simulink model "My_gfm_battery_sil_1_BS_4_2"  (R2018b)
settings: Solver=ode23t  StartTime=0.0  StopTime=30  MaxStep=1e-4  RelTol=1e-3
PreLoadFcn:
  | modelDir = fileparts(get_param(bdroot,'FileName'));
  | 
  | load_system(fullfile(modelDir,'controls_element_lib.slx'));
  | load_system(fullfile(modelDir,'test_sequence_lib.slx'));
InitFcn:
  | close all;
  | clear all;
  | clc;
  | 
  | % frequency nominals
  | F_NOM = 60;
  | W_NOM = 2 * pi * F_NOM;
  | 
  | % base values relative to inverter
  | % --------------------------------
  | VLL_INV_NOM = 480;
  | P_INV_NOM = 1e6;
  | Q_INV_NOM = 0.5e6;
  | S_INV_NOM = sqrt(P_INV_NOM^2 + Q_INV_NOM^2);
  | 
  | I_INV_BASE = S_INV_NOM/(sqrt(3)*VLL_INV_NOM);
  | Z_INV_BASE = VLL_INV_NOM^2/S_INV_NOM;
  | L_INV_BASE = Z_INV_BASE / W_NOM;
  | C_INV_BASE = 1 / (Z_INV_BASE * W_NOM);
  | 
  | % nominal ratings for power system model
  | % --------------------------------------
  | INVERTER_COUNT = 100;
  | 
  | VLV_NOM = VLL_INV_NOM;
  | VMV_NOM = 35e3;
  | VHV_NOM = 230e3;
  | S_PLANT = INVERTER_COUNT * S_INV_NOM;
  | 
  | N_GSU = VHV_NOM/VMV_NOM;
  | N_MVT = VMV_NOM/VLV_NOM;
  | 
  | I_LV_BASE = S_PLANT/(sqrt(3)*VLV_NOM);
  | I_MV_BASE = S_PLANT/(sqrt(3)*VMV_NOM);
  | I_HV_BASE = S_PLANT/(sqrt(3)*VHV_NOM);
  | 
  | Z_LV_BASE = VLV_NOM^2/S_PLANT;
  | Z_MV_BASE = VMV_NOM^2/S_PLANT;
  | Z_HV_BASE = VHV_NOM^2/S_PLANT;
  | 
  | L_LV_BASE = Z_LV_BASE / W_NOM;
  | L_MV_BASE = Z_MV_BASE / W_NOM;
  | L_HV_BASE = Z_HV_BASE / W_NOM;
  | C_LV_BASE = 1 / (Z_LV_BASE * W_NOM);
  | C_MV_BASE = 1 / (Z_MV_BASE * W_NOM);
  | C_HV_BASE = 1 / (Z_HV_BASE * W_NOM);
undefined symbols (not defined in the file): j
libraries: simulink x54, test_sequence_lib x9, controls_element_lib x7
(part 6 of 6)

== system My_gfm_battery_sil_1_BS_4_2/My Inverter Controller /My_machineModel_Other Exciter/power analyzer ==
  iac : Inport
  vac : Inport  Port=2
  Demux1 : Demux  Outputs=3
  Demux2 : Demux  Outputs=3
  Gain3 : Gain  Gain=1 / sqrt(3)
  Product{,1..3} (4 alike) : Product
  Sum of Elements : Sum  Inputs=+
  Sum2 : Sum  Inputs=|+-
  Sum3 : Sum  Inputs=|+-
  Sum4 : Sum  Inputs=|+-
  Sum5 : Sum  Inputs=+++
  P : Outport  VectorParamsAs1DForOutWhenUnconnected=on
  Q : Outport  Port=2  VectorParamsAs1DForOutWhenUnconnected=on
  wires:
  Product/1 -> Sum of Elements/1
  Sum of Elements/1 -> P/1  "P"
  Gain3/1 -> Q/1  "Q"
  Demux1/1 -> Product2/2  "ia"
  Demux2/1 -> Sum2/1, Sum4/2
  Sum2/1 -> Product1/1  "vab"
  Sum5/1 -> Gain3/1
  Sum3/1 -> Product2/1  "vbc"
  iac/1 -> Demux1/1, Product/1
  vac/1 -> Product/2, Demux2/1
  Demux1/2 -> Product3/2  "ib"
  Demux1/3 -> Product1/2  "ic"
  Demux2/3 -> Sum3/2, Sum4/1
  Demux2/2 -> Sum2/2, Sum3/1
  Product3/1 -> Sum5/2
  Sum4/1 -> Product3/1  "vca"
  Product2/1 -> Sum5/3
  Product1/1 -> Sum5/1

== system My_gfm_battery_sil_1_BS_4_2/My Inverter Controller /My_machineModel_Other Exciter/rotor model ==
  p_mechanical : Inport
  p_electrical : Inport  Port=2
  Constant : Constant  Value=nominalFrequency
  HPF (wDamperDecoupler) : TransferFcn  Commented=on  Numerator=[0.3 0]  Denominator=[0.3 1]
  HPF (wDamperDecoupler) 1 : Subsystem
  Integrator1 : Integrator  LimitOutput=on  UpperSaturationLimit=5  LowerSaturationLimit=-5
  Sum : Sum  Inputs=++|
  Sum2 : Sum  Inputs=|+-
  Sum3 : Sum  Inputs=|+-
  k_damp : Gain  Gain=kDamper*SRated
  k_inertia : Gain  Gain=(nominalFrequency/2)/(inertialConstant*SRated)
  oscillator_3ph : Subsystem
  osc[3] : Outport  VectorParamsAs1DForOutWhenUnconnected=on
  f_rotor : Outport  Port=2  VectorParamsAs1DForOutWhenUnconnected=on
  wires:
  Constant/1 -> Sum/1
  Sum/1 -> oscillator_3ph/1(f), f_rotor/1
  k_damp/1 -> Sum2/2
  Integrator1/1 -> HPF (wDamperDecoupler) 1/1(in), Sum/2
  p_mechanical/1 -> Sum3/1
  Sum3/1 -> Sum2/1
  p_electrical/1 -> Sum3/2
  HPF (wDamperDecoupler) 1/1(out) -> k_damp/1
  oscillator_3ph/1(osc[3]) -> osc[3]/1
  k_inertia/1 -> Integrator1/1
  Sum2/1 -> k_inertia/1

== system My_gfm_battery_sil_1_BS_4_2/My Inverter Controller /My_machineModel_Other Exciter/voltage analyzer ==
  osc[3] : Inport
  v_terminal : Inport  Port=2
  Complex to Magnitude-Angle : ComplexToMagnitudeAngle
  Complex to Real-Imag : ComplexToRealImag
  Conj : Math  Operator=conj  SaturateOnIntegerOverflow=on
  LPF : Subsystem
  "LPF " : Subsystem
  Product1 : Product
  Product2 : Product
  Real-Imag to Complex1 : RealImagToComplex
  Sum of Elements1 : Sum  Inputs=+
  Sum of Elements2 : Sum  Inputs=+
  Terminator : Terminator
  over_sqrt(3) : Gain  Gain=1/sqrt(3)
  over_sqrt(3)1 : Gain  Gain=1/sqrt(3)
  sqrt(2) : Gain  Gain=sqrt(2)
  Vd : Outport  VectorParamsAs1DForOutWhenUnconnected=on
  Vq : Outport  Port=2  VectorParamsAs1DForOutWhenUnconnected=on
  Vt_Mag : Outport  Port=3  VectorParamsAs1DForOutWhenUnconnected=on
  wires:
  "LPF "/1(Out) -> Real-Imag to Complex1/2, Vq/1  "Vq"
  osc[3]/1 -> Conj/1
  LPF/1(Out) -> Real-Imag to Complex1/1, Vd/1  "Vd"
  over_sqrt(3)1/1 -> LPF/1(In)
  over_sqrt(3)/1 -> "LPF "/1(In)
  Complex to Real-Imag/1 -> Product2/1
  Complex to Real-Imag/2 -> Product1/1
  Sum of Elements2/1 -> over_sqrt(3)1/1
  v_terminal/1 -> Product2/2, Product1/2
  Product1/1 -> Sum of Elements1/1
  Sum of Elements1/1 -> over_sqrt(3)/1
  sqrt(2)/1 -> Complex to Real-Imag/1
  Conj/1 -> sqrt(2)/1
  Product2/1 -> Sum of Elements2/1
  Complex to Magnitude-Angle/1 -> Vt_Mag/1  "Vt"
  Real-Imag to Complex1/1 -> Complex to Magnitude-Angle/1  "Vd"
  Complex to Magnitude-Angle/2 -> Terminator/1

== system My_gfm_battery_sil_1_BS_4_2/My Inverter Controller /modesAndProtection_A/hardware_protection ==
  vdc : Inport
  Clear Timer : Subsystem  mask{T_STEP=1e-3, TIMEOUT=dcTripClearTimeout}
      mask prompts: T_STEP "Time step"
  Compare To Constant1 : simulink/Logic and Bit Operations/Compare To Constant  relop=<  const=dcUndervotlageThreshold  OutDataTypeStr=boolean
  Compare To Constant2 : simulink/Logic and Bit Operations/Compare To Constant  relop=>  const=dcOvervotlageThreshold  OutDataTypeStr=boolean
  NOT : Logic  Operator=NOT  IconShape=distinctive  AllPortsSameDT=off  OutDataTypeStr=boolean
  OR : Logic  Operator=OR  IconShape=distinctive  AllPortsSameDT=off  OutDataTypeStr=boolean
  Zero-Order Hold1 : ZeroOrderHold  SampleTime=200e-6
  all_clear : Outport  VectorParamsAs1DForOutWhenUnconnected=on
  wires:
  NOT/1 -> all_clear/1
  Zero-Order Hold1/1 -> Compare To Constant2/1, Compare To Constant1/1
  Compare To Constant2/1 -> OR/1  "dcOV"
  Clear Timer/1(out) -> NOT/1
  OR/1 -> Clear Timer/1(in)
  Compare To Constant1/1 -> OR/2  "dcUV"
  vdc/1 -> Zero-Order Hold1/1

== system My_gfm_battery_sil_1_BS_4_2/Plant controller (simplified example)1/LVRT_foldback/LPF ==
  in : Inport
  1/0.01 : Gain  Gain=1/0.01
  Integrator : Integrator
  Sum3 : Sum  Inputs=|+-
  out : Outport  VectorParamsAs1DForOutWhenUnconnected=on
  wires:
  Integrator/1 -> out/1, Sum3/2
  Sum3/1 -> 1/0.01/1
  in/1 -> Sum3/1
  1/0.01/1 -> Integrator/1

== system My_gfm_battery_sil_1_BS_4_2/Plant controller (simplified example)1/LVRT_foldback/assymmetric filter ==
  in : Inport
  Gain1 : Gain  Gain=1/0.01
  Integrator : Integrator
  Saturation1 : Saturate  UpperLimit=0.05 * 1  LowerLimit=-1 * 1
  Sum3 : Sum  Inputs=|+-
  out : Outport  VectorParamsAs1DForOutWhenUnconnected=on
  wires:
  Integrator/1 -> out/1, Sum3/2
  Sum3/1 -> Saturation1/1
  in/1 -> Sum3/1
  Gain1/1 -> Integrator/1
  Saturation1/1 -> Gain1/1

== system My_gfm_battery_sil_1_BS_4_2/Plant controller (simplified example)1/Meter/PLL-analog ==
  note: cos x - j sin x
      | cos (x-120) - j (sin x -120)
      | cos (x+120) - j (sin x +120)
  note: cos x + j sin x
      | cos (x-120) + j (sin x -120)
      | cos (x+120) + j (sin x +120)
  note: -sin x
      |  -sin (x -120)
      |  -sin (x +120)
  note: cos x + j sin x
      | cos (x-120) + j (sin x -120)
      | cos (x+120) + j (sin x +120)
  ref : Inport
  Complex to Real-Imag : ComplexToRealImag
  Conj : Math  Operator=conj  SaturateOnIntegerOverflow=on
  Gain : Gain  Gain=3
  Gain2 : Gain  Gain=30
  Integrator : Integrator  LimitOutput=on  UpperSaturationLimit=5  LowerSaturationLimit=-5
  Product2 : Product
  Saturation : Saturate  UpperLimit=5  LowerLimit=-5
  Sum of Elements : Sum  Inputs=+
  Sum1 : Sum  Inputs=|++
  Sum2 : Sum  Inputs=|++
  Terminator : Terminator
  Transfer Fcn : TransferFcn  Denominator=[0.02 1]
  fnom : Constant  Value=60
  oscillator_3ph : Subsystem
  freq : Outport  VectorParamsAs1DForOutWhenUnconnected=on
  osc : Outport  Port=2  VectorParamsAs1DForOutWhenUnconnected=on
  wires:
  Gain2/1 -> Integrator/1
  Integrator/1 -> Sum2/2
  Sum2/1 -> Sum1/1
  fnom/1 -> Sum1/2
  Product2/1 -> Sum of Elements/1
  Transfer Fcn/1 -> Gain/1, Gain2/1
  Saturation/1 -> Sum2/1
  Gain/1 -> Saturation/1
  Sum1/1 -> oscillator_3ph/1(f), freq/1
  ref/1 -> Product2/1
  Sum of Elements/1 -> Transfer Fcn/1
  Conj/1 -> Complex to Real-Imag/1
  Complex to Real-Imag/1 -> Terminator/1
  Complex to Real-Imag/2 -> Product2/2
  oscillator_3ph/1(osc[3]) -> osc/1, Conj/1

== system My_gfm_battery_sil_1_BS_4_2/Plant controller (simplified example)1/VoltVAr/LPF ==
  in : Inport
  1/0.05 : Gain  Gain=1/0.05
  Integrator : Integrator
  Sum3 : Sum  Inputs=|+-
  out : Outport  VectorParamsAs1DForOutWhenUnconnected=on
  wires:
  Integrator/1 -> out/1, Sum3/2
  Sum3/1 -> 1/0.05/1
  in/1 -> Sum3/1
  1/0.05/1 -> Integrator/1

== system My_gfm_battery_sil_1_BS_4_2/Plant controller (simplified example)1/VoltVAr/LPF1 ==
  in : Inport
  1/0.05 : Gain  Gain=1/0.05
  1/0.1 : Gain
  Integrator : Integrator
  Saturation : Saturate  UpperLimit=inf  LowerLimit=0
  Saturation1 : Saturate  UpperLimit=0  LowerLimit=-inf
  Sum : Sum  Inputs=|++
  Sum3 : Sum  Inputs=|+-
  out : Outport  VectorParamsAs1DForOutWhenUnconnected=on
  wires:
  Integrator/1 -> out/1, Sum3/2
  Sum3/1 -> 1/0.1/1, 1/0.05/1
  in/1 -> Sum3/1
  1/0.05/1 -> Saturation/1
  Sum/1 -> Integrator/1
  1/0.1/1 -> Saturation1/1
  Saturation/1 -> Sum/1
  Saturation1/1 -> Sum/2

== system My_gfm_battery_sil_1_BS_4_2/Plant controller (simplified example)2/LVRT_foldback/LPF ==
  in : Inport
  1/0.01 : Gain  Gain=1/0.01
  Integrator : Integrator
  Sum3 : Sum  Inputs=|+-
  out : Outport  VectorParamsAs1DForOutWhenUnconnected=on
  wires:
  Integrator/1 -> out/1, Sum3/2
  Sum3/1 -> 1/0.01/1
  in/1 -> Sum3/1
  1/0.01/1 -> Integrator/1

== system My_gfm_battery_sil_1_BS_4_2/Plant controller (simplified example)2/LVRT_foldback/assymmetric filter ==
  in : Inport
  Gain1 : Gain  Gain=1/0.01
  Integrator : Integrator
  Saturation1 : Saturate  UpperLimit=0.05 * 1  LowerLimit=-1 * 1
  Sum3 : Sum  Inputs=|+-
  out : Outport  VectorParamsAs1DForOutWhenUnconnected=on
  wires:
  Integrator/1 -> out/1, Sum3/2
  Sum3/1 -> Saturation1/1
  in/1 -> Sum3/1
  Gain1/1 -> Integrator/1
  Saturation1/1 -> Gain1/1

== system My_gfm_battery_sil_1_BS_4_2/Plant controller (simplified example)2/Meter/PLL-analog ==
  note: cos x - j sin x
      | cos (x-120) - j (sin x -120)
      | cos (x+120) - j (sin x +120)
  note: cos x + j sin x
      | cos (x-120) + j (sin x -120)
      | cos (x+120) + j (sin x +120)
  note: -sin x
      |  -sin (x -120)
      |  -sin (x +120)
  note: cos x + j sin x
      | cos (x-120) + j (sin x -120)
      | cos (x+120) + j (sin x +120)
  ref : Inport
  en : Inport  Port=2
  Complex to Real-Imag : ComplexToRealImag
  Conj : Math  Operator=conj  SaturateOnIntegerOverflow=on
  Gain : Gain  Gain=3
  Gain2 : Gain  Gain=30
  Integrator : Integrator  ExternalReset=level  LimitOutput=on  UpperSaturationLimit=5  LowerSaturationLimit=-5
  Logical Operator : Logic  Operator=NOT  IconShape=distinctive  AllPortsSameDT=off  OutDataTypeStr=boolean
  Product2 : Product
  Saturation : Saturate  UpperLimit=5  LowerLimit=-5
  Sum of Elements : Sum  Inputs=+
  Sum1 : Sum  Inputs=|++
  Sum2 : Sum  Inputs=|++
  Terminator : Terminator
  Transfer Fcn : TransferFcn  Denominator=[0.02 1]
  fnom : Constant  Value=60
  oscillator_3ph : Subsystem
  freq : Outport  VectorParamsAs1DForOutWhenUnconnected=on
  osc : Outport  Port=2  VectorParamsAs1DForOutWhenUnconnected=on
  wires:
  Gain2/1 -> Integrator/1
  Integrator/1 -> Sum2/2
  Sum2/1 -> Sum1/1
  fnom/1 -> Sum1/2
  Product2/1 -> Sum of Elements/1
  Transfer Fcn/1 -> Gain/1, Gain2/1
  Saturation/1 -> Sum2/1
  Gain/1 -> Saturation/1
  Sum1/1 -> oscillator_3ph/1(f), freq/1
  ref/1 -> Product2/1
  Sum of Elements/1 -> Transfer Fcn/1
  Conj/1 -> Complex to Real-Imag/1
  Complex to Real-Imag/1 -> Terminator/1
  Complex to Real-Imag/2 -> Product2/2
  oscillator_3ph/1(osc[3]) -> osc/1, Conj/1
  en/1 -> Logical Operator/1
  Logical Operator/1 -> Integrator/2

== system My_gfm_battery_sil_1_BS_4_2/Plant controller (simplified example)2/Sync/LPF ==
  In : Inport
  1/0.02 : Gain  Gain=1/0.02
  Integrator : Integrator
  Sum3 : Sum  Inputs=|+-
  Out : Outport  VectorParamsAs1DForOutWhenUnconnected=on
  wires:
  Integrator/1 -> Out/1, Sum3/2
  Sum3/1 -> 1/0.02/1
  In/1 -> Sum3/1
  1/0.02/1 -> Integrator/1

== system My_gfm_battery_sil_1_BS_4_2/Plant controller (simplified example)2/Sync/LPF1 ==
  In : Inport
  1/0.02 : Gain  Gain=1/0.02
  Integrator : Integrator
  Sum3 : Sum  Inputs=|+-
  Out : Outport  VectorParamsAs1DForOutWhenUnconnected=on
  wires:
  Integrator/1 -> Out/1, Sum3/2
  Sum3/1 -> 1/0.02/1
  In/1 -> Sum3/1
  1/0.02/1 -> Integrator/1

== system My_gfm_battery_sil_1_BS_4_2/Plant controller (simplified example)2/VoltVAr/LPF ==
  in : Inport
  1/0.05 : Gain  Gain=1/0.05
  Integrator : Integrator
  Sum3 : Sum  Inputs=|+-
  out : Outport  VectorParamsAs1DForOutWhenUnconnected=on
  wires:
  Integrator/1 -> out/1, Sum3/2
  Sum3/1 -> 1/0.05/1
  in/1 -> Sum3/1
  1/0.05/1 -> Integrator/1

== system My_gfm_battery_sil_1_BS_4_2/Plant controller (simplified example)2/VoltVAr/LPF1 ==
  in : Inport
  1/0.05 : Gain  Gain=1/0.05
  1/0.1 : Gain
  Integrator : Integrator
  Saturation : Saturate  UpperLimit=inf  LowerLimit=0
  Saturation1 : Saturate  UpperLimit=0  LowerLimit=-inf
  Sum : Sum  Inputs=|++
  Sum3 : Sum  Inputs=|+-
  out : Outport  VectorParamsAs1DForOutWhenUnconnected=on
  wires:
  Integrator/1 -> out/1, Sum3/2
  Sum3/1 -> 1/0.1/1, 1/0.05/1
  in/1 -> Sum3/1
  1/0.05/1 -> Saturation/1
  Sum/1 -> Integrator/1
  1/0.1/1 -> Saturation1/1
  Saturation/1 -> Sum/1
  Saturation1/1 -> Sum/2

== system My_gfm_battery_sil_1_BS_4_2/My Inverter Controller /My_acMonitor_A/Analyzer_V/complex_LPF ==
  note: This was needed because Simulink complains when using transfer functions directly on arrays or complex numbers.
  In1 : Inport
  Complex to Real-Imag : ComplexToRealImag
  Gain2 : Gain  Gain=1/tau
  Gain3 : Gain  Gain=1/tau
  Integrator : Integrator
  Integrator1 : Integrator
  Real-Imag to Complex : RealImagToComplex
  Sum : Sum  Inputs=|+-
  Sum1 : Sum  Inputs=|+-
  Out1 : Outport  VectorParamsAs1DForOutWhenUnconnected=on
  wires:
  Real-Imag to Complex/1 -> Out1/1
  In1/1 -> Complex to Real-Imag/1
  Complex to Real-Imag/1 -> Sum/1
  Integrator/1 -> Real-Imag to Complex/1, Sum/2
  Sum1/1 -> Gain3/1
  Complex to Real-Imag/2 -> Sum1/1
  Gain2/1 -> Integrator/1
  Sum/1 -> Gain2/1
  Integrator1/1 -> Sum1/2, Real-Imag to Complex/2
  Gain3/1 -> Integrator1/1

== system My_gfm_battery_sil_1_BS_4_2/My Inverter Controller /My_acMonitor_A/Analyzer_V1/complex_LPF ==
  note: This was needed because Simulink complains when using transfer functions directly on arrays or complex numbers.
  In1 : Inport
  Complex to Real-Imag : ComplexToRealImag
  Gain2 : Gain  Gain=1/tau
  Gain3 : Gain  Gain=1/tau
  Integrator : Integrator
  Integrator1 : Integrator
  Real-Imag to Complex : RealImagToComplex
  Sum : Sum  Inputs=|+-
  Sum1 : Sum  Inputs=|+-
  Out1 : Outport  VectorParamsAs1DForOutWhenUnconnected=on
  wires:
  Real-Imag to Complex/1 -> Out1/1
  In1/1 -> Complex to Real-Imag/1
  Complex to Real-Imag/1 -> Sum/1
  Integrator/1 -> Real-Imag to Complex/1, Sum/2
  Sum1/1 -> Gain3/1
  Complex to Real-Imag/2 -> Sum1/1
  Gain2/1 -> Integrator/1
  Sum/1 -> Gain2/1
  Integrator1/1 -> Sum1/2, Real-Imag to Complex/2
  Gain3/1 -> Integrator1/1

== system My_gfm_battery_sil_1_BS_4_2/My Inverter Controller /My_acMonitor_A/PLL_3ph/oscillator_3ph ==
  f : Inport
  Cos : Trigonometry  Operator=cos
  Gain : Gain  Gain=2*pi
  Integrator : Integrator
  Real-Imag to Complex : RealImagToComplex
  Sin : Trigonometry
  Sum1 : Sum  Inputs=|++
  phase_shift : Constant  Value=[0 -1/3 -2/3]
  osc[3] : Outport  VectorParamsAs1DForOutWhenUnconnected=on
  wires:
  Sum1/1 -> Gain/1
  phase_shift/1 -> Sum1/2
  Sin/1 -> Real-Imag to Complex/2
  Integrator/1 -> Sum1/1
  Gain/1 -> Sin/1, Cos/1
  Cos/1 -> Real-Imag to Complex/1
  Real-Imag to Complex/1 -> osc[3]/1
  f/1 -> Integrator/1

== system My_gfm_battery_sil_1_BS_4_2/My Inverter Controller /My_currentLimiting_B/Current_foldback1/LPF  ==
  In : Inport
  1/0.01 : Gain  Gain=1/0.01
  Integrator : Integrator
  Sum3 : Sum  Inputs=|+-
  Out : Outport  VectorParamsAs1DForOutWhenUnconnected=on
  wires:
  Integrator/1 -> Out/1, Sum3/2
  Sum3/1 -> 1/0.01/1
  In/1 -> Sum3/1
  1/0.01/1 -> Integrator/1

== system My_gfm_battery_sil_1_BS_4_2/My Inverter Controller /My_machineModel_A1/excitation/LPF ==
  In : Inport
  Integrator : Integrator
  Sum3 : Sum  Inputs=|+-
  wExciter : Gain  Gain=wExciter
  Out : Outport  VectorParamsAs1DForOutWhenUnconnected=on
  wires:
  Integrator/1 -> Out/1, Sum3/2
  Sum3/1 -> wExciter/1
  In/1 -> Sum3/1
  wExciter/1 -> Integrator/1

== system My_gfm_battery_sil_1_BS_4_2/My Inverter Controller /My_machineModel_A1/excitation/assymmetric filter1 ==
  note: The saturation block is configured to cause a rapid rise, but much slow drop in output.
  in : Inport
  Gain1 : Gain  Gain=2
  Integrator : Integrator
  Saturation1 : Saturate  UpperLimit=VllRated  LowerLimit=-0.02 * VllRated
  Sum3 : Sum  Inputs=|+-
  out : Outport  VectorParamsAs1DForOutWhenUnconnected=on
  wires:
  Saturation1/1 -> Integrator/1
  Gain1/1 -> Saturation1/1
  in/1 -> Sum3/1
  Sum3/1 -> Gain1/1
  Integrator/1 -> Sum3/2, out/1

== system My_gfm_battery_sil_1_BS_4_2/My Inverter Controller /My_machineModel_A1/excitation/modulator ==
  cmd : Inport
  osc : Inport  Port=2
  Complex to Real-Imag : ComplexToRealImag
  Complex to Real-Imag1 : ComplexToRealImag
  Gain : Gain  Gain=sqrt(2)
  Product1 : Product
  Product2 : Product
  Sum1 : Sum  Inputs=|+-
  ref : Outport  VectorParamsAs1DForOutWhenUnconnected=on
  wires:
  osc/1 -> Gain/1
  Complex to Real-Imag/1 -> Product2/2
  Product2/1 -> Sum1/1
  Sum1/1 -> ref/1  "i"
  Gain/1 -> Complex to Real-Imag/1
  Complex to Real-Imag/2 -> Product1/2
  Product1/1 -> Sum1/2
  cmd/1 -> Complex to Real-Imag1/1
  Complex to Real-Imag1/1 -> Product2/1
  Complex to Real-Imag1/2 -> Product1/1

== system My_gfm_battery_sil_1_BS_4_2/My Inverter Controller /My_machineModel_A1/governer/LPF(DamperDecoupler) limited  ==
  In : Inport
  1/tau_damp : Gain  Gain=1/0.3
  Integrator : Integrator  LimitOutput=on  UpperSaturationLimit=1.2*SRated  LowerSaturationLimit=-1.2*SRated
  Sum3 : Sum  Inputs=|+-
  Out : Outport  VectorParamsAs1DForOutWhenUnconnected=on
  wires:
  Integrator/1 -> Out/1, Sum3/2
  Sum3/1 -> 1/tau_damp/1
  In/1 -> Sum3/1
  1/tau_damp/1 -> Integrator/1

== system My_gfm_battery_sil_1_BS_4_2/My Inverter Controller /My_machineModel_A1/governer/synchronizer ==
  note: Why?
  note: Big Range?
  note: prevent it from acting during typical faults
  note: Prevent loss of sync at low voltage events, using asym filter to traget long extended low voltage events
  note: Keeps the machine spining in synchronize while machine is disabled, disabling the machine means
  note: Why?
  Vq : Inport
  Vt : Inport  Port=2
  machine_enabled : Inport  Port=3
  Constant : Constant
  Gain : Gain  Gain=SRated
  Gain2 : Gain  Gain=1/VllRated
  HPF : Subsystem
  Product1 : Product
  Saturation : Saturate  UpperLimit=1  LowerLimit=0
  Sum : Sum  Inputs=|++
  Sum2 : Sum  Inputs=|+-
  Switch : Switch  Criteria=u2 > Threshold
  Transfer Fcn : TransferFcn  Commented=on  Numerator=[(2 * pi * 50) 0]  Denominator=[1, (2*pi*50)]
  assymmetric filter1 : Subsystem
  gain : Gain  Gain=2*pi*50
  kFastSync : Gain
  kSync : Gain  Gain=20
  pSyncLimit : Saturate  UpperLimit=3  LowerLimit=-3
  syncFadeGain : Gain  Gain=4
  syncFadeThreshold : Constant  Value=0.2
  to_pu : Gain  Gain=1 / VllRated
  p_sync_pu : Outport  VectorParamsAs1DForOutWhenUnconnected=on
  wires:
  to_pu/1 -> Sum2/2
  Vt/1 -> assymmetric filter1/1(in)
  assymmetric filter1/1(out) -> to_pu/1
  pSyncLimit/1 -> Gain/1
  kSync/1 -> Sum/1
  Sum/1 -> pSyncLimit/1
  Product1/1 -> p_sync_pu/1
  Constant/1 -> Switch/3
  Sum2/1 -> syncFadeGain/1
  machine_enabled/1 -> Switch/2
  syncFadeGain/1 -> Saturation/1
  Saturation/1 -> Switch/1
  syncFadeThreshold/1 -> Sum2/1
  Switch/1 -> Product1/2
  Gain2/1 -> kFastSync/1, kSync/1
  Vq/1 -> Gain2/1
  Gain/1 -> Product1/1  "p_sync"
  kFastSync/1 -> HPF/1(in)
  HPF/1(out) -> gain/1
  gain/1 -> Sum/2

== system My_gfm_battery_sil_1_BS_4_2/My Inverter Controller /My_machineModel_A1/governer1/LPF(DamperDecoupler) - limited ==
  In1 : Inport
  Integrator : Integrator  LimitOutput=on  UpperSaturationLimit=1.2*SRated  LowerSaturationLimit=-1.2*SRated
  Sum3 : Sum  Inputs=|+-
  wDamperDecoupler : Gain  Gain=1/0.3
  Out1 : Outport  VectorParamsAs1DForOutWhenUnconnected=on
  wires:
  Integrator/1 -> Out1/1, Sum3/2
  Sum3/1 -> wDamperDecoupler/1
  wDamperDecoupler/1 -> Integrator/1
  In1/1 -> Sum3/1

== system My_gfm_battery_sil_1_BS_4_2/My Inverter Controller /My_machineModel_A1/governer1/LPF(DamperDecoupler) limited 1 ==
  In : Inport
  1/tau_damp : Gain  Gain=1/0.3
  Integrator : Integrator  LimitOutput=on  UpperSaturationLimit=1.2*SRated  LowerSaturationLimit=-1.2*SRated
  Sum3 : Sum  Inputs=|+-
  Out : Outport  VectorParamsAs1DForOutWhenUnconnected=on
  wires:
  Integrator/1 -> Out/1, Sum3/2
  Sum3/1 -> 1/tau_damp/1
  In/1 -> Sum3/1
  1/tau_damp/1 -> Integrator/1

== system My_gfm_battery_sil_1_BS_4_2/My Inverter Controller /My_machineModel_A1/governer1/synchronizer ==
  note: Why?
  note: Big Range?
  note: prevent it from acting during typical faults
  note: Prevent loss of sync at low voltage events, using asym filter to traget long extended low voltage events
  note: Keeps the machine spining in synchronize while machine is disabled, disabling the machine means
  note: Why?
  note: Should be sqrt(Vd^2 + Vq^2) ?
  Vq : Inport
  Vd : Inport  Port=2
  machine_enabled : Inport  Port=3
  Constant : Constant
  Gain : Gain  Gain=SRated
  Gain2 : Gain  Gain=1/VllRated
  HPF : Subsystem
  Product1 : Product
  Saturation : Saturate  UpperLimit=1  LowerLimit=0
  Sum : Sum  Inputs=|++
  Sum2 : Sum  Inputs=|+-
  Switch : Switch  Criteria=u2 > Threshold
  Transfer Fcn : TransferFcn  Commented=on  Numerator=[(2 * pi * 50) 0]  Denominator=[1, (2*pi*50)]
  assymmetric filter1 : Subsystem
  gain : Gain  Gain=2*pi*50
  kFastSync : Gain
  kSync : Gain  Gain=20
  pSyncLimit : Saturate  UpperLimit=3  LowerLimit=-3
  syncFadeGain : Gain  Gain=4
  syncFadeThreshold : Constant  Value=0.2
  to_pu : Gain  Gain=1 / VllRated
  p_sync_pu : Outport  VectorParamsAs1DForOutWhenUnconnected=on
  wires:
  to_pu/1 -> Sum2/2
  Vd/1 -> assymmetric filter1/1(in)
  assymmetric filter1/1(out) -> to_pu/1
  pSyncLimit/1 -> Gain/1
  kSync/1 -> Sum/1
  Sum/1 -> pSyncLimit/1
  Product1/1 -> p_sync_pu/1
  Constant/1 -> Switch/3
  Sum2/1 -> syncFadeGain/1
  machine_enabled/1 -> Switch/2
  syncFadeGain/1 -> Saturation/1
  Saturation/1 -> Switch/1
  syncFadeThreshold/1 -> Sum2/1
  Switch/1 -> Product1/2
  Gain2/1 -> kFastSync/1, kSync/1
  Vq/1 -> Gain2/1
  Gain/1 -> Product1/1  "p_sync"
  kFastSync/1 -> HPF/1(in)
  HPF/1(out) -> gain/1
  gain/1 -> Sum/2

== system My_gfm_battery_sil_1_BS_4_2/My Inverter Controller /My_machineModel_A1/rotor model/HPF (wDamperDecoupler) 1 ==
  in : Inport
  1/tau_damp : Gain  Gain=1/0.3
  Integrator : Integrator
  Sum : Sum  Inputs=|+-
  out : Outport  VectorParamsAs1DForOutWhenUnconnected=on
  wires:
  Sum/1 -> out/1, 1/tau_damp/1
  in/1 -> Sum/1
  Integrator/1 -> Sum/2
  1/tau_damp/1 -> Integrator/1

== system My_gfm_battery_sil_1_BS_4_2/My Inverter Controller /My_machineModel_A1/rotor model/oscillator_3ph ==
  f : Inport
  Cos : Trigonometry  Operator=cos
  Gain : Gain  Gain=2*pi
  Integrator : Integrator
  Real-Imag to Complex : RealImagToComplex
  Sin : Trigonometry
  Sum1 : Sum  Inputs=|++
  phase_shift : Constant  Value=[0 -1/3 -2/3]
  osc[3] : Outport  VectorParamsAs1DForOutWhenUnconnected=on
  wires:
  f/1 -> Integrator/1
  Real-Imag to Complex/1 -> osc[3]/1
  Cos/1 -> Real-Imag to Complex/1
  Gain/1 -> Cos/1, Sin/1
  Integrator/1 -> Sum1/1
  Sin/1 -> Real-Imag to Complex/2
  phase_shift/1 -> Sum1/2
  Sum1/1 -> Gain/1

== system My_gfm_battery_sil_1_BS_4_2/My Inverter Controller /My_machineModel_Other Exciter/AVR/LPF ==
  In : Inport
  1/tauMeas : Gain  Gain=1/tauMeas
  Integrator : Integrator
  Sum3 : Sum  Inputs=|+-
  Out : Outport  VectorParamsAs1DForOutWhenUnconnected=on
  wires:
  Integrator/1 -> Out/1, Sum3/2
  Sum3/1 -> 1/tauMeas/1
  In/1 -> Sum3/1
  1/tauMeas/1 -> Integrator/1

== system My_gfm_battery_sil_1_BS_4_2/My Inverter Controller /My_machineModel_Other Exciter/AVR/V LPF ==
  In : Inport
  1/tpv : Gain  Gain=1/tpv
  Integrator : Integrator
  Sum3 : Sum  Inputs=|+-
  Out : Outport  VectorParamsAs1DForOutWhenUnconnected=on
  wires:
  Integrator/1 -> Out/1, Sum3/2
  Sum3/1 -> 1/tpv/1
  In/1 -> Sum3/1
  1/tpv/1 -> Integrator/1

== system My_gfm_battery_sil_1_BS_4_2/My Inverter Controller /My_machineModel_Other Exciter/AVR/assymmetric filter ==
  note: The saturation block is configured to cause a rapid rise, but much slow drop in output.
  in : Inport
  en : Inport  Port=2
  Gain1 : Gain  Gain=1/tauBkSt
  Integrator : Integrator  ExternalReset=level
  Logical Operator : Logic  Operator=NOT  IconShape=distinctive  AllPortsSameDT=off  OutDataTypeStr=boolean
  Saturation1 : Saturate  UpperLimit=VllRated  LowerLimit=-0.02 * VllRated
  Sum3 : Sum  Inputs=|+-
  out : Outport  VectorParamsAs1DForOutWhenUnconnected=on
  wires:
  Saturation1/1 -> Integrator/1
  Gain1/1 -> Saturation1/1
  in/1 -> Sum3/1
  Sum3/1 -> Gain1/1
  Integrator/1 -> Sum3/2, out/1
  en/1 -> Logical Operator/1
  Logical Operator/1 -> Integrator/2

== system My_gfm_battery_sil_1_BS_4_2/My Inverter Controller /My_machineModel_Other Exciter/AVR1/LPF ==
  In : Inport
  1/tauMeas : Gain  Gain=1/tauMeas
  Integrator : Integrator
  Sum3 : Sum  Inputs=|+-
  Out : Outport  VectorParamsAs1DForOutWhenUnconnected=on
  wires:
  Integrator/1 -> Out/1, Sum3/2
  Sum3/1 -> 1/tauMeas/1
  In/1 -> Sum3/1
  1/tauMeas/1 -> Integrator/1

== system My_gfm_battery_sil_1_BS_4_2/My Inverter Controller /My_machineModel_Other Exciter/AVR1/V LPF ==
  In : Inport
  1/tpv : Gain  Gain=1/tpv
  Integrator : Integrator
  Sum3 : Sum  Inputs=|+-
  Out : Outport  VectorParamsAs1DForOutWhenUnconnected=on
  wires:
  Integrator/1 -> Out/1, Sum3/2
  Sum3/1 -> 1/tpv/1
  In/1 -> Sum3/1
  1/tpv/1 -> Integrator/1

== system My_gfm_battery_sil_1_BS_4_2/My Inverter Controller /My_machineModel_Other Exciter/AVR1/assymmetric filter ==
  note: The saturation block is configured to cause a rapid rise, but much slow drop in output.
  in : Inport
  Gain1 : Gain  Gain=1/tauBkSt
  Integrator : Integrator
  Saturation1 : Saturate  UpperLimit=VllRated  LowerLimit=-0.02 * VllRated
  Sum3 : Sum  Inputs=|+-
  out : Outport  VectorParamsAs1DForOutWhenUnconnected=on
  wires:
  Saturation1/1 -> Integrator/1
  Gain1/1 -> Saturation1/1
  in/1 -> Sum3/1
  Sum3/1 -> Gain1/1
  Integrator/1 -> Sum3/2, out/1

== system My_gfm_battery_sil_1_BS_4_2/My Inverter Controller /My_machineModel_Other Exciter/Exciter/LPF ==
  In : Inport
  Integrator : Integrator
  Sum3 : Sum  Inputs=|+-
  wExciter : Gain  Gain=wExciter
  Out : Outport  VectorParamsAs1DForOutWhenUnconnected=on
  wires:
  Integrator/1 -> Out/1, Sum3/2
  Sum3/1 -> wExciter/1
  In/1 -> Sum3/1
  wExciter/1 -> Integrator/1

== system My_gfm_battery_sil_1_BS_4_2/My Inverter Controller /My_machineModel_Other Exciter/Exciter/modulator ==
  cmd : Inport
  osc : Inport  Port=2
  Complex to Real-Imag : ComplexToRealImag
  Complex to Real-Imag1 : ComplexToRealImag
  Gain : Gain  Gain=sqrt(2)
  Product1 : Product
  Product2 : Product
  Sum1 : Sum  Inputs=|+-
  ref : Outport  VectorParamsAs1DForOutWhenUnconnected=on
  wires:
  osc/1 -> Gain/1
  Complex to Real-Imag/1 -> Product2/2
  Product2/1 -> Sum1/1
  Sum1/1 -> ref/1  "i"
  Gain/1 -> Complex to Real-Imag/1
  Complex to Real-Imag/2 -> Product1/2
  Product1/1 -> Sum1/2
  cmd/1 -> Complex to Real-Imag1/1
  Complex to Real-Imag1/1 -> Product2/1
  Complex to Real-Imag1/2 -> Product1/1

== system My_gfm_battery_sil_1_BS_4_2/My Inverter Controller /My_machineModel_Other Exciter/governer/LPF(DamperDecoupler) limited  ==
  In : Inport
  Constant : Constant  Value=1/tau_damp
  Constant1 : Constant  Value=wGoverner
  Integrator : Integrator  LimitOutput=on  UpperSaturationLimit=1.2*SRated  LowerSaturationLimit=-1.2*SRated
  MinMax : MinMax  Inputs=2
  Product : Product
  Sum3 : Sum  Inputs=|+-
  Out : Outport  VectorParamsAs1DForOutWhenUnconnected=on
  wires:
  Integrator/1 -> Out/1, Sum3/2
  Sum3/1 -> Product/2
  In/1 -> Sum3/1
  Product/1 -> Integrator/1
  MinMax/1 -> Product/1
  Constant/1 -> MinMax/1
  Constant1/1 -> MinMax/2

== system My_gfm_battery_sil_1_BS_4_2/My Inverter Controller /My_machineModel_Other Exciter/governer/synchronizer ==
  note: Big Range?
  note: prevent it from acting during typical faults
  note: Prevent loss of sync at low voltage events, using asym filter to traget long extended low voltage events
  note: Keeps the machine spining in synchronize while machine is disabled, disabling the machine means
  note: Why?
  Vq : Inport
  Vt : Inport  Port=2
  machine_enabled : Inport  Port=3
  Constant : Constant
  Gain : Gain  Gain=SRated
  Gain2 : Gain  Gain=1/VllRated
  "HPF " : Subsystem
  Product1 : Product
  Saturation : Saturate  UpperLimit=1  LowerLimit=0
  Sum : Sum  Inputs=|++
  Sum2 : Sum  Inputs=|+-
  Switch : Switch  Criteria=u2 > Threshold
  assymmetric filter1 : Subsystem
  gain : Gain  Gain=wSync
  kFastSync : Gain  Gain=kpFastSync
  kSync : Gain  Gain=kpSync
  pSyncLimit : Saturate  UpperLimit=3  LowerLimit=-3
  syncFadeGain : Gain  Gain=kpSyncFade
  syncFadeThreshold : Constant  Value=SyncFadeThres
  to_pu : Gain  Gain=1 / VllRated
  p_sync_pu : Outport  VectorParamsAs1DForOutWhenUnconnected=on
  wires:
  to_pu/1 -> Sum2/2
  Vt/1 -> assymmetric filter1/1(in)
  assymmetric filter1/1(out) -> to_pu/1
  pSyncLimit/1 -> Gain/1
  kSync/1 -> Sum/1
  Sum/1 -> pSyncLimit/1
  Product1/1 -> p_sync_pu/1
  Constant/1 -> Switch/3
  Sum2/1 -> syncFadeGain/1
  machine_enabled/1 -> Switch/2
  syncFadeGain/1 -> Saturation/1
  Saturation/1 -> Switch/1
  syncFadeThreshold/1 -> Sum2/1
  Switch/1 -> Product1/2
  Gain2/1 -> kFastSync/1, kSync/1
  Vq/1 -> Gain2/1
  Gain/1 -> Product1/1  "p_sync"
  kFastSync/1 -> "HPF "/1(in)
  "HPF "/1(out) -> gain/1
  gain/1 -> Sum/2

== system My_gfm_battery_sil_1_BS_4_2/My Inverter Controller /My_machineModel_Other Exciter/rotor model/HPF (wDamperDecoupler) 1 ==
  in : Inport
  1/tau_damp : Gain  Gain=1/tau_damp
  Integrator : Integrator
  Sum : Sum  Inputs=|+-
  out : Outport  VectorParamsAs1DForOutWhenUnconnected=on
  wires:
  Sum/1 -> out/1, 1/tau_damp/1
  in/1 -> Sum/1
  Integrator/1 -> Sum/2
  1/tau_damp/1 -> Integrator/1

== system My_gfm_battery_sil_1_BS_4_2/My Inverter Controller /My_machineModel_Other Exciter/rotor model/oscillator_3ph ==
  f : Inport
  Cos : Trigonometry  Operator=cos
  Gain : Gain  Gain=2*pi
  Integrator : Integrator
  Real-Imag to Complex : RealImagToComplex
  Sin : Trigonometry
  Sum1 : Sum  Inputs=|++
  phase_shift : Constant  Value=[0 -1/3 -2/3]
  osc[3] : Outport  VectorParamsAs1DForOutWhenUnconnected=on
  wires:
  f/1 -> Integrator/1
  Real-Imag to Complex/1 -> osc[3]/1
  Cos/1 -> Real-Imag to Complex/1
  Gain/1 -> Cos/1, Sin/1
  Integrator/1 -> Sum1/1
  Sin/1 -> Real-Imag to Complex/2
  phase_shift/1 -> Sum1/2
  Sum1/1 -> Gain/1

== system My_gfm_battery_sil_1_BS_4_2/My Inverter Controller /My_machineModel_Other Exciter/voltage analyzer/LPF ==
  In : Inport
  1/tauMeas : Gain  Gain=1/tauMeas
  Integrator : Integrator
  Sum3 : Sum  Inputs=|+-
  Out : Outport  VectorParamsAs1DForOutWhenUnconnected=on
  wires:
  Integrator/1 -> Out/1, Sum3/2
  Sum3/1 -> 1/tauMeas/1
  In/1 -> Sum3/1
  1/tauMeas/1 -> Integrator/1

== system My_gfm_battery_sil_1_BS_4_2/My Inverter Controller /My_machineModel_Other Exciter/voltage analyzer/LPF  ==
  In : Inport
  1/tauMeas : Gain  Gain=1/tauMeas
  Integrator : Integrator
  Sum3 : Sum  Inputs=|+-
  Out : Outport  VectorParamsAs1DForOutWhenUnconnected=on
  wires:
  Integrator/1 -> Out/1, Sum3/2
  Sum3/1 -> 1/tauMeas/1
  In/1 -> Sum3/1
  1/tauMeas/1 -> Integrator/1

== system My_gfm_battery_sil_1_BS_4_2/My Inverter Controller /modesAndProtection_A/hardware_protection/Clear Timer ==
  in : Inport
  Constant : Constant  Value=T_STEP
  Constant1 : Constant  Value=0
  Constant2 : Constant  Value=TIMEOUT
  Min2 : MinMax  Function=max  Inputs=2
  Relational Operator : RelationalOperator  Operator=>  OutDataTypeStr=boolean  RndMeth=Simplest
  Sum2 : Sum  Inputs=|-+
  Switch : Switch  Criteria=u2 > Threshold
  Unit Delay : UnitDelay  SampleTime=T_STEP
  out : Outport  VectorParamsAs1DForOutWhenUnconnected=on
  wires:
  Relational Operator/1 -> out/1
  Switch/1 -> Unit Delay/1
  in/1 -> Switch/2
  Unit Delay/1 -> Sum2/2
  Constant2/1 -> Switch/1
  Min2/1 -> Switch/3
  Constant/1 -> Sum2/1
  Constant1/1 -> Relational Operator/2, Min2/2
  Sum2/1 -> Min2/1, Relational Operator/1

== system My_gfm_battery_sil_1_BS_4_2/Plant controller (simplified example)1/Meter/PLL-analog/oscillator_3ph ==
  f : Inport
  Cos : Trigonometry  Operator=cos
  Gain : Gain  Gain=2*pi
  Integrator : Integrator
  Real-Imag to Complex : RealImagToComplex
  Sin : Trigonometry
  Sum1 : Sum  Inputs=|++
  phase_shift : Constant  Value=[0 -1/3 -2/3]
  osc[3] : Outport  VectorParamsAs1DForOutWhenUnconnected=on
  wires:
  Sum1/1 -> Gain/1
  phase_shift/1 -> Sum1/2
  Sin/1 -> Real-Imag to Complex/2
  Integrator/1 -> Sum1/1
  Gain/1 -> Sin/1, Cos/1
  Cos/1 -> Real-Imag to Complex/1
  Real-Imag to Complex/1 -> osc[3]/1
  f/1 -> Integrator/1

== system My_gfm_battery_sil_1_BS_4_2/Plant controller (simplified example)2/Meter/PLL-analog/oscillator_3ph ==
  f : Inport
  Cos : Trigonometry  Operator=cos
  Gain : Gain  Gain=2*pi
  Integrator : Integrator
  Real-Imag to Complex : RealImagToComplex
  Sin : Trigonometry
  Sum1 : Sum  Inputs=|++
  phase_shift : Constant  Value=[0 -1/3 -2/3]
  osc[3] : Outport  VectorParamsAs1DForOutWhenUnconnected=on
  wires:
  Sum1/1 -> Gain/1
  phase_shift/1 -> Sum1/2
  Sin/1 -> Real-Imag to Complex/2
  Integrator/1 -> Sum1/1
  Gain/1 -> Sin/1, Cos/1
  Cos/1 -> Real-Imag to Complex/1
  Real-Imag to Complex/1 -> osc[3]/1
  f/1 -> Integrator/1

== system My_gfm_battery_sil_1_BS_4_2/My Inverter Controller /My_machineModel_A1/governer/synchronizer/HPF ==
  in : Inport
  1/tau : Gain  Gain=2*pi*50
  Integrator : Integrator
  Sum : Sum  Inputs=|+-
  out : Outport  VectorParamsAs1DForOutWhenUnconnected=on
  wires:
  Sum/1 -> out/1, 1/tau/1
  in/1 -> Sum/1
  Integrator/1 -> Sum/2
  1/tau/1 -> Integrator/1

== system My_gfm_battery_sil_1_BS_4_2/My Inverter Controller /My_machineModel_A1/governer/synchronizer/assymmetric filter1 ==
  note: The saturation block is configured to cause a rapid rise, but much slow drop in output.
  in : Inport
  Gain1 : Gain  Gain=2
  Integrator : Integrator
  Saturation1 : Saturate  UpperLimit=VllRated  LowerLimit=-0.02 * VllRated
  Sum3 : Sum  Inputs=|+-
  out : Outport  VectorParamsAs1DForOutWhenUnconnected=on
  wires:
  Integrator/1 -> out/1, Sum3/2
  Sum3/1 -> Gain1/1
  in/1 -> Sum3/1
  Gain1/1 -> Saturation1/1
  Saturation1/1 -> Integrator/1

== system My_gfm_battery_sil_1_BS_4_2/My Inverter Controller /My_machineModel_A1/governer1/synchronizer/HPF ==
  in : Inport
  1/tau : Gain  Gain=2*pi*50
  Integrator : Integrator
  Sum : Sum  Inputs=|+-
  out : Outport  VectorParamsAs1DForOutWhenUnconnected=on
  wires:
  Sum/1 -> out/1, 1/tau/1
  in/1 -> Sum/1
  Integrator/1 -> Sum/2
  1/tau/1 -> Integrator/1

== system My_gfm_battery_sil_1_BS_4_2/My Inverter Controller /My_machineModel_A1/governer1/synchronizer/assymmetric filter1 ==
  note: The saturation block is configured to cause a rapid rise, but much slow drop in output.
  in : Inport
  Gain1 : Gain  Gain=2
  Integrator : Integrator
  Saturation1 : Saturate  UpperLimit=VllRated  LowerLimit=-0.02 * VllRated
  Sum3 : Sum  Inputs=|+-
  out : Outport  VectorParamsAs1DForOutWhenUnconnected=on
  wires:
  Integrator/1 -> out/1, Sum3/2
  Sum3/1 -> Gain1/1
  in/1 -> Sum3/1
  Gain1/1 -> Saturation1/1
  Saturation1/1 -> Integrator/1

== system My_gfm_battery_sil_1_BS_4_2/My Inverter Controller /My_machineModel_Other Exciter/governer/synchronizer/HPF  ==
  in : Inport
  Integrator : Integrator
  Sum : Sum  Inputs=|+-
  wSync : Gain  Gain=wSync
  out : Outport  VectorParamsAs1DForOutWhenUnconnected=on
  wires:
  Sum/1 -> out/1, wSync/1
  in/1 -> Sum/1
  Integrator/1 -> Sum/2
  wSync/1 -> Integrator/1

== system My_gfm_battery_sil_1_BS_4_2/My Inverter Controller /My_machineModel_Other Exciter/governer/synchronizer/assymmetric filter1 ==
  note: The saturation block is configured to cause a rapid rise, but much slow drop in output.
  in : Inport
  Gain1 : Gain  Gain=1/tauBkSt
  Integrator : Integrator
  Saturation1 : Saturate  UpperLimit=VllRated  LowerLimit=-0.02 * VllRated
  Sum3 : Sum  Inputs=|+-
  out : Outport  VectorParamsAs1DForOutWhenUnconnected=on
  wires:
  Integrator/1 -> out/1, Sum3/2
  Sum3/1 -> Gain1/1
  in/1 -> Sum3/1
  Gain1/1 -> Saturation1/1
  Saturation1/1 -> Integrator/1
